simulink model "MMC_phase_hackathon_consensus_PWM_JABBAR_20260927"  (R2024b)
settings: Solver=FixedStepDiscrete  StartTime=t_init_sim  StopTime=sim_time  FixedStep=Ts  RelTol=1e-3
values from neighbouring files (symbols this model uses):
  a = 1    [script_MMC_phase_hackathon_consensus_PWM_JABBAR_20260927.m]
  C1low1_active = 1    [script_MMC_phase_hackathon_consensus_PWM_JABBAR_20260927.m]
  C2low1_active = 1    [script_MMC_phase_hackathon_consensus_PWM_JABBAR_20260927.m]
  C_bus = 4400e-6    (= 0.0044)    [script_MMC_phase_hackathon_consensus_PWM_JABBAR_20260927.m]
  C_M_extra = C_m-twist_high_side_C    [script_MMC_phase_hackathon_consensus_PWM_JABBAR_20260927.m]
  f0 = 50    [script_MMC_phase_hackathon_consensus_PWM_JABBAR_20260927.m]
  feeder_current_lower_rate_limit = -10    [script_MMC_phase_hackathon_consensus_PWM_JABBAR_20260927.m]    (also in twist_parameters.m = -500)
  feeder_current_tab = [0.328 0.217 0.162 0.132 0.109 0.094 0.083 0.075 0.068 0.062 0.058 0.054 ... (42 elements, 14x3)]    [feeder_current.mat]
  feeder_current_upper_rate_limit = 0.386/(20e-3)    (= 19.3)    [twist_parameters.m]
  is6VExternallySupplied = true    [script_MMC_phase_hackathon_consensus_PWM_JABBAR_20260927.m]
  isFeederJumperOpen = true    [script_MMC_phase_hackathon_consensus_PWM_JABBAR_20260927.m]
  L_arm = 100e-3    (= 0.1)    [script_MMC_phase_hackathon_consensus_PWM_JABBAR_20260927.m]
  m = 1    [script_MMC_phase_hackathon_consensus_PWM_JABBAR_20260927.m]
  power_losses = false    [script_MMC_phase_hackathon_consensus_PWM_JABBAR_20260927.m]
  R = 30    [script_MMC_phase_hackathon_consensus_PWM_JABBAR_20260927.m]
  R_arm = 0.2    [script_MMC_phase_hackathon_consensus_PWM_JABBAR_20260927.m]
  source_V = 0    [script_MMC_phase_hackathon_consensus_PWM_JABBAR_20260927.m]
  time_charge = 0.1    [script_MMC_phase_hackathon_consensus_PWM_JABBAR_20260927.m]
  time_decharge = 1.5    [script_MMC_phase_hackathon_consensus_PWM_JABBAR_20260927.m]
  Ts = 5e-7    (= 5e-07)    [script_MMC_phase_hackathon_consensus_PWM_JABBAR_20260927.m]
  twist_data_acquisition_delay = 50e-9    (= 5e-08)    [script_MMC_phase_hackathon_consensus_PWM_JABBAR_20260927.m]    (also in twist_parameters.m)
  twist_data_sampling_period = 1/twist_freq_data_sampling    (= 5e-05)    [script_MMC_phase_hackathon_consensus_PWM_JABBAR_20260927.m]    (also in twist_parameters.m)
  twist_dead_time = 200e-9    (= 2e-07)    [twist_parameters.m]
  twist_freq_switching = 200e3    (= 200000)    [twist_parameters.m]
  twist_high_side_adc_R = 1/(1/2e6 + 1/2e6 + 1/(330e3+5.6e3))    (= 251272.836178)    [twist_parameters.m]
  twist_high_side_C = 33e-6*4 + 4.7e-6*12    (= 0.0001884)    [twist_parameters.m]
  twist_high_side_feeder_R = 47e3+4.7e3    (= 51700)    [twist_parameters.m]
  twist_high_side_rC = 0.1    [twist_parameters.m]
  twist_low_side_adc_R = 150e3+470    (= 150470)    [twist_parameters.m]
  twist_low_side_C_ceramic = 3*4.7e-6    (= 1.41e-05)    [twist_parameters.m]
  twist_low_side_C_electrolytic = 47e-6    (= 4.7e-05)    [twist_parameters.m]
  twist_low_side_L = 33e-6    (= 3.3e-05)    [twist_parameters.m]
  twist_low_side_rC = 700e-3    (= 0.7)    [twist_parameters.m]
  twist_low_side_rL = 20e-3    (= 0.02)    [twist_parameters.m]
  twist_R_VCC = (tau_VCC/twist_high_side_C  - twist_high_side_rC)/(1-(tau_VCC/twist_high_side_C - twist_high_side_rC)/R_parallel)    (= 1110.74997822)    [twist_parameters.m]
  VDC = 48    [script_MMC_phase_hackathon_consensus_PWM_JABBAR_20260927.m]
undefined symbols (not defined in the file or in its folder): C_SM, feeder_current, gcbh, sps_rtmsupport, twist_low_side_lC
libraries: spsSeriesRLCBranchLib x135, spsTriangleGeneratorLib x60, spsMosfetLib x60, spsCurrentMeasurementLib x43, spsVoltageMeasurementLib x35, spsControlledCurrentSourceLib x30, spsDiodeLib x22, spsIdealSwitchLib x20, spsControlledVoltageSourceLib x1, spsGroundLib x1, spspowerguiLib x1
(part 17 of 19)

== system MMC_phase_hackathon_consensus_PWM_JABBAR_20260927/ /Subsystem/Subsystem1/Hardware M5/HRTimA_1/PWM Generator (2-Level)/Sampling/Sync Asymmetrical/Sample & Hold ==
  In : Inport
  Enable : EnablePort
  Out : Outport  VectorParamsAs1DForOutWhenUnconnected=off
  wires:
  In/1 -> Out/1

== system MMC_phase_hackathon_consensus_PWM_JABBAR_20260927/ /Subsystem/Subsystem1/Hardware M5/HRTimA_1/PWM Generator (2-Level)/Sampling/Sync Natural/Sync_NaturalSampling ==
  Uref : Inport  Interpolate=off
  wt : Inport  Port=2  Interpolate=off
  Gain1 : Gain  Gain=2/pi  SaturateOnIntegerOverflow=on  OutDataTypeStr=Inherit: Same as input  ParamDataTypeStr=Inherit: Same as input
  Gain4 : Gain  Gain=nF  SaturateOnIntegerOverflow=on  OutDataTypeStr=Inherit: Same as input  ParamDataTypeStr=Inherit: Same as input
  Trigonometric Function : Trigonometry  Operator=asin
  Trigonometric Function3 : Trigonometry
  Uref* : Outport  VectorParamsAs1DForOutWhenUnconnected=off
  Cr : Outport  Port=2  VectorParamsAs1DForOutWhenUnconnected=off
  wires:
  wt/1 -> Gain4/1
  Gain1/1 -> Cr/1
  Trigonometric Function/1 -> Gain1/1
  Trigonometric Function3/1 -> Trigonometric Function/1
  Gain4/1 -> Trigonometric Function3/1
  Uref/1 -> Uref*/1

== system MMC_phase_hackathon_consensus_PWM_JABBAR_20260927/ /Subsystem/Subsystem1/Hardware M5/HRTimA_1/PWM Generator (2-Level)/Sampling/Sync Symmetrical/Sync_SymmetricalSampling ==
  Uref : Inport  Interpolate=off
  wt : Inport  Port=2  Interpolate=off
  Add : Sum
  Constant3 : Constant
  Gain1 : Gain  Gain=2/pi  SaturateOnIntegerOverflow=on  OutDataTypeStr=Inherit: Same as input  ParamDataTypeStr=Inherit: Same as input
  Gain4 : Gain  Gain=nF  SaturateOnIntegerOverflow=on  OutDataTypeStr=Inherit: Same as input  ParamDataTypeStr=Inherit: Same as input
  Hit Crossing : HitCross  HitCrossingOffset=1e-9  HitCrossingDirection=falling
  Sample & Hold : Subsystem
  Trigonometric Function : Trigonometry  Operator=asin
  Trigonometric Function3 : Trigonometry
  Uref* : Outport  VectorParamsAs1DForOutWhenUnconnected=off
  Cr : Outport  Port=2  VectorParamsAs1DForOutWhenUnconnected=off
  wires:
  wt/1 -> Gain4/1
  Gain1/1 -> Cr/1, Add/1
  Trigonometric Function/1 -> Gain1/1
  Trigonometric Function3/1 -> Trigonometric Function/1
  Gain4/1 -> Trigonometric Function3/1
  Add/1 -> Hit Crossing/1
  Constant3/1 -> Add/2
  Hit Crossing/1 -> Sample & Hold/Enable
  Uref/1 -> Sample & Hold/1(In)
  Sample & Hold/1(Out) -> Uref*/1

== system MMC_phase_hackathon_consensus_PWM_JABBAR_20260927/ /Subsystem/Subsystem1/Hardware M5/HRTimA_1/PWM Generator (2-Level)/Sampling/Unsync Asymmetrical/Unsync_AsymmetricalSampling ==
  Uref : Inport  Interpolate=off
  Triangle Generator : spsTriangleGeneratorLib/Triangle Generator  Freq=sps.Fc  Phase=sps.Pc  Ts=Ts
  Zero-Order Hold : ZeroOrderHold  SampleTime=sps.SampleTimeZOH_AsymSampling
  Uref* : Outport  VectorParamsAs1DForOutWhenUnconnected=off
  Cr : Outport  Port=2  VectorParamsAs1DForOutWhenUnconnected=off
  wires:
  Triangle Generator/1 -> Cr/1
  Uref/1 -> Zero-Order Hold/1
  Zero-Order Hold/1 -> Uref*/1

== system MMC_phase_hackathon_consensus_PWM_JABBAR_20260927/ /Subsystem/Subsystem1/Hardware M5/HRTimA_1/PWM Generator (2-Level)/Sampling/Unsync Natural/Unsync_NaturalSampling ==
  Uref : Inport  Interpolate=off
  Triangle Generator : spsTriangleGeneratorLib/Triangle Generator  Freq=sps.Fc  Phase=sps.Pc  Ts=Ts
  Uref* : Outport  VectorParamsAs1DForOutWhenUnconnected=off
  Cr : Outport  Port=2  VectorParamsAs1DForOutWhenUnconnected=off
  wires:
  Triangle Generator/1 -> Cr/1
  Uref/1 -> Uref*/1

== system MMC_phase_hackathon_consensus_PWM_JABBAR_20260927/ /Subsystem/Subsystem1/Hardware M5/HRTimA_1/PWM Generator (2-Level)/Sampling/Unsync Symmetrical/Unsync_SymmetricalSampling ==
  Uref : Inport  Interpolate=off
  Triangle Generator : spsTriangleGeneratorLib/Triangle Generator  Freq=sps.Fc  Phase=sps.Pc  Ts=Ts
  Zero-Order Hold : ZeroOrderHold  SampleTime=sps.SampleTimeZOH_SymSampling
  Uref* : Outport  VectorParamsAs1DForOutWhenUnconnected=off
  Cr : Outport  Port=2  VectorParamsAs1DForOutWhenUnconnected=off
  wires:
  Triangle Generator/1 -> Cr/1
  Uref/1 -> Zero-Order Hold/1
  Zero-Order Hold/1 -> Uref*/1

== system MMC_phase_hackathon_consensus_PWM_JABBAR_20260927/ /Subsystem/Subsystem1/Hardware M5/HRTimA_2/PWM Generator (2-Level)/Sampling/Sync Asymmetrical/Sample & Hold ==
  In : Inport
  Enable : EnablePort
  Out : Outport  VectorParamsAs1DForOutWhenUnconnected=off
  wires:
  In/1 -> Out/1

== system MMC_phase_hackathon_consensus_PWM_JABBAR_20260927/ /Subsystem/Subsystem1/Hardware M5/HRTimA_2/PWM Generator (2-Level)/Sampling/Sync Natural/Sync_NaturalSampling ==
  Uref : Inport  Interpolate=off
  wt : Inport  Port=2  Interpolate=off
  Gain1 : Gain  Gain=2/pi  SaturateOnIntegerOverflow=on  OutDataTypeStr=Inherit: Same as input  ParamDataTypeStr=Inherit: Same as input
  Gain4 : Gain  Gain=nF  SaturateOnIntegerOverflow=on  OutDataTypeStr=Inherit: Same as input  ParamDataTypeStr=Inherit: Same as input
  Trigonometric Function : Trigonometry  Operator=asin
  Trigonometric Function3 : Trigonometry
  Uref* : Outport  VectorParamsAs1DForOutWhenUnconnected=off
  Cr : Outport  Port=2  VectorParamsAs1DForOutWhenUnconnected=off
  wires:
  wt/1 -> Gain4/1
  Gain1/1 -> Cr/1
  Trigonometric Function/1 -> Gain1/1
  Trigonometric Function3/1 -> Trigonometric Function/1
  Gain4/1 -> Trigonometric Function3/1
  Uref/1 -> Uref*/1

== system MMC_phase_hackathon_consensus_PWM_JABBAR_20260927/ /Subsystem/Subsystem1/Hardware M5/HRTimA_2/PWM Generator (2-Level)/Sampling/Sync Symmetrical/Sync_SymmetricalSampling ==
  Uref : Inport  Interpolate=off
  wt : Inport  Port=2  Interpolate=off
  Add : Sum
  Constant3 : Constant
  Gain1 : Gain  Gain=2/pi  SaturateOnIntegerOverflow=on  OutDataTypeStr=Inherit: Same as input  ParamDataTypeStr=Inherit: Same as input
  Gain4 : Gain  Gain=nF  SaturateOnIntegerOverflow=on  OutDataTypeStr=Inherit: Same as input  ParamDataTypeStr=Inherit: Same as input
  Hit Crossing : HitCross  HitCrossingOffset=1e-9  HitCrossingDirection=falling
  Sample & Hold : Subsystem
  Trigonometric Function : Trigonometry  Operator=asin
  Trigonometric Function3 : Trigonometry
  Uref* : Outport  VectorParamsAs1DForOutWhenUnconnected=off
  Cr : Outport  Port=2  VectorParamsAs1DForOutWhenUnconnected=off
  wires:
  wt/1 -> Gain4/1
  Gain1/1 -> Cr/1, Add/1
  Trigonometric Function/1 -> Gain1/1
  Trigonometric Function3/1 -> Trigonometric Function/1
  Gain4/1 -> Trigonometric Function3/1
  Add/1 -> Hit Crossing/1
  Constant3/1 -> Add/2
  Hit Crossing/1 -> Sample & Hold/Enable
  Uref/1 -> Sample & Hold/1(In)
  Sample & Hold/1(Out) -> Uref*/1

== system MMC_phase_hackathon_consensus_PWM_JABBAR_20260927/ /Subsystem/Subsystem1/Hardware M5/HRTimA_2/PWM Generator (2-Level)/Sampling/Unsync Asymmetrical/Unsync_AsymmetricalSampling ==
  Uref : Inport  Interpolate=off
  Triangle Generator : spsTriangleGeneratorLib/Triangle Generator  Freq=sps.Fc  Phase=sps.Pc  Ts=Ts
  Zero-Order Hold : ZeroOrderHold  SampleTime=sps.SampleTimeZOH_AsymSampling
  Uref* : Outport  VectorParamsAs1DForOutWhenUnconnected=off
  Cr : Outport  Port=2  VectorParamsAs1DForOutWhenUnconnected=off
  wires:
  Triangle Generator/1 -> Cr/1
  Uref/1 -> Zero-Order Hold/1
  Zero-Order Hold/1 -> Uref*/1

== system MMC_phase_hackathon_consensus_PWM_JABBAR_20260927/ /Subsystem/Subsystem1/Hardware M5/HRTimA_2/PWM Generator (2-Level)/Sampling/Unsync Natural/Unsync_NaturalSampling ==
  Uref : Inport  Interpolate=off
  Triangle Generator : spsTriangleGeneratorLib/Triangle Generator  Freq=sps.Fc  Phase=sps.Pc  Ts=Ts
  Uref* : Outport  VectorParamsAs1DForOutWhenUnconnected=off
  Cr : Outport  Port=2  VectorParamsAs1DForOutWhenUnconnected=off
  wires:
  Triangle Generator/1 -> Cr/1
  Uref/1 -> Uref*/1

== system MMC_phase_hackathon_consensus_PWM_JABBAR_20260927/ /Subsystem/Subsystem1/Hardware M5/HRTimA_2/PWM Generator (2-Level)/Sampling/Unsync Symmetrical/Unsync_SymmetricalSampling ==
  Uref : Inport  Interpolate=off
  Triangle Generator : spsTriangleGeneratorLib/Triangle Generator  Freq=sps.Fc  Phase=sps.Pc  Ts=Ts
  Zero-Order Hold : ZeroOrderHold  SampleTime=sps.SampleTimeZOH_SymSampling
  Uref* : Outport  VectorParamsAs1DForOutWhenUnconnected=off
  Cr : Outport  Port=2  VectorParamsAs1DForOutWhenUnconnected=off
  wires:
  Triangle Generator/1 -> Cr/1
  Uref/1 -> Zero-Order Hold/1
  Zero-Order Hold/1 -> Uref*/1

== system MMC_phase_hackathon_consensus_PWM_JABBAR_20260927/ /Subsystem/Subsystem/Hardware M1/HRTimA_1/PWM Generator (2-Level)/Sampling/Sync Symmetrical/Sync_SymmetricalSampling/Sample & Hold ==
  In : Inport
  Enable : EnablePort
  Out : Outport  VectorParamsAs1DForOutWhenUnconnected=off
  wires:
  In/1 -> Out/1

== system MMC_phase_hackathon_consensus_PWM_JABBAR_20260927/ /Subsystem/Subsystem/Hardware M1/HRTimA_2/PWM Generator (2-Level)/Sampling/Sync Symmetrical/Sync_SymmetricalSampling/Sample & Hold ==
  In : Inport
  Enable : EnablePort
  Out : Outport  VectorParamsAs1DForOutWhenUnconnected=off
  wires:
  In/1 -> Out/1

== system MMC_phase_hackathon_consensus_PWM_JABBAR_20260927/ /Subsystem/Subsystem/Hardware M2/HRTimA_1/PWM Generator (2-Level)/Sampling/Sync Symmetrical/Sync_SymmetricalSampling/Sample & Hold ==
  In : Inport
  Enable : EnablePort
  Out : Outport  VectorParamsAs1DForOutWhenUnconnected=off
  wires:
  In/1 -> Out/1

== system MMC_phase_hackathon_consensus_PWM_JABBAR_20260927/ /Subsystem/Subsystem/Hardware M2/HRTimA_2/PWM Generator (2-Level)/Sampling/Sync Symmetrical/Sync_SymmetricalSampling/Sample & Hold ==
  In : Inport
  Enable : EnablePort
  Out : Outport  VectorParamsAs1DForOutWhenUnconnected=off
  wires:
  In/1 -> Out/1

== system MMC_phase_hackathon_consensus_PWM_JABBAR_20260927/ /Subsystem/Subsystem/Hardware M3/HRTimA_1/PWM Generator (2-Level)/Sampling/Sync Symmetrical/Sync_SymmetricalSampling/Sample & Hold ==
  In : Inport
  Enable : EnablePort
  Out : Outport  VectorParamsAs1DForOutWhenUnconnected=off
  wires:
  In/1 -> Out/1

== system MMC_phase_hackathon_consensus_PWM_JABBAR_20260927/ /Subsystem/Subsystem/Hardware M3/HRTimA_2/PWM Generator (2-Level)/Sampling/Sync Symmetrical/Sync_SymmetricalSampling/Sample & Hold ==
  In : Inport
  Enable : EnablePort
  Out : Outport  VectorParamsAs1DForOutWhenUnconnected=off
  wires:
  In/1 -> Out/1

== system MMC_phase_hackathon_consensus_PWM_JABBAR_20260927/ /Subsystem/Subsystem/Hardware M4/HRTimA_1/PWM Generator (2-Level)/Sampling/Sync Symmetrical/Sync_SymmetricalSampling/Sample & Hold ==
  In : Inport
  Enable : EnablePort
  Out : Outport  VectorParamsAs1DForOutWhenUnconnected=off
  wires:
  In/1 -> Out/1

== system MMC_phase_hackathon_consensus_PWM_JABBAR_20260927/ /Subsystem/Subsystem/Hardware M4/HRTimA_2/PWM Generator (2-Level)/Sampling/Sync Symmetrical/Sync_SymmetricalSampling/Sample & Hold ==
  In : Inport
  Enable : EnablePort
  Out : Outport  VectorParamsAs1DForOutWhenUnconnected=off
  wires:
  In/1 -> Out/1

== system MMC_phase_hackathon_consensus_PWM_JABBAR_20260927/ /Subsystem/Subsystem/Hardware M5/HRTimA_1/PWM Generator (2-Level)/Sampling/Sync Symmetrical/Sync_SymmetricalSampling/Sample & Hold ==
  In : Inport
  Enable : EnablePort
  Out : Outport  VectorParamsAs1DForOutWhenUnconnected=off
  wires:
  In/1 -> Out/1

== system MMC_phase_hackathon_consensus_PWM_JABBAR_20260927/ /Subsystem/Subsystem/Hardware M5/HRTimA_2/PWM Generator (2-Level)/Sampling/Sync Symmetrical/Sync_SymmetricalSampling/Sample & Hold ==
  In : Inport
  Enable : EnablePort
  Out : Outport  VectorParamsAs1DForOutWhenUnconnected=off
  wires:
  In/1 -> Out/1

== system MMC_phase_hackathon_consensus_PWM_JABBAR_20260927/ /Subsystem/Subsystem1/Hardware M1/HRTimA_1/PWM Generator (2-Level)/Sampling/Sync Symmetrical/Sync_SymmetricalSampling/Sample & Hold ==
  In : Inport
  Enable : EnablePort
  Out : Outport  VectorParamsAs1DForOutWhenUnconnected=off
  wires:
  In/1 -> Out/1

== system MMC_phase_hackathon_consensus_PWM_JABBAR_20260927/ /Subsystem/Subsystem1/Hardware M1/HRTimA_2/PWM Generator (2-Level)/Sampling/Sync Symmetrical/Sync_SymmetricalSampling/Sample & Hold ==
  In : Inport
  Enable : EnablePort
  Out : Outport  VectorParamsAs1DForOutWhenUnconnected=off
  wires:
  In/1 -> Out/1

== system MMC_phase_hackathon_consensus_PWM_JABBAR_20260927/ /Subsystem/Subsystem1/Hardware M2/HRTimA_1/PWM Generator (2-Level)/Sampling/Sync Symmetrical/Sync_SymmetricalSampling/Sample & Hold ==
  In : Inport
  Enable : EnablePort
  Out : Outport  VectorParamsAs1DForOutWhenUnconnected=off
  wires:
  In/1 -> Out/1

== system MMC_phase_hackathon_consensus_PWM_JABBAR_20260927/ /Subsystem/Subsystem1/Hardware M2/HRTimA_2/PWM Generator (2-Level)/Sampling/Sync Symmetrical/Sync_SymmetricalSampling/Sample & Hold ==
  In : Inport
  Enable : EnablePort
  Out : Outport  VectorParamsAs1DForOutWhenUnconnected=off
  wires:
  In/1 -> Out/1

== system MMC_phase_hackathon_consensus_PWM_JABBAR_20260927/ /Subsystem/Subsystem1/Hardware M3/HRTimA_1/PWM Generator (2-Level)/Sampling/Sync Symmetrical/Sync_SymmetricalSampling/Sample & Hold ==
  In : Inport
  Enable : EnablePort
  Out : Outport  VectorParamsAs1DForOutWhenUnconnected=off
  wires:
  In/1 -> Out/1

== system MMC_phase_hackathon_consensus_PWM_JABBAR_20260927/ /Subsystem/Subsystem1/Hardware M3/HRTimA_2/PWM Generator (2-Level)/Sampling/Sync Symmetrical/Sync_SymmetricalSampling/Sample & Hold ==
  In : Inport
  Enable : EnablePort
  Out : Outport  VectorParamsAs1DForOutWhenUnconnected=off
  wires:
  In/1 -> Out/1

== system MMC_phase_hackathon_consensus_PWM_JABBAR_20260927/ /Subsystem/Subsystem1/Hardware M4/HRTimA_1/PWM Generator (2-Level)/Sampling/Sync Symmetrical/Sync_SymmetricalSampling/Sample & Hold ==
  In : Inport
  Enable : EnablePort
  Out : Outport  VectorParamsAs1DForOutWhenUnconnected=off
  wires:
  In/1 -> Out/1

== system MMC_phase_hackathon_consensus_PWM_JABBAR_20260927/ /Subsystem/Subsystem1/Hardware M4/HRTimA_2/PWM Generator (2-Level)/Sampling/Sync Symmetrical/Sync_SymmetricalSampling/Sample & Hold ==
  In : Inport
  Enable : EnablePort
  Out : Outport  VectorParamsAs1DForOutWhenUnconnected=off
  wires:
  In/1 -> Out/1

== system MMC_phase_hackathon_consensus_PWM_JABBAR_20260927/ /Subsystem/Subsystem1/Hardware M5/HRTimA_1/PWM Generator (2-Level)/Sampling/Sync Symmetrical/Sync_SymmetricalSampling/Sample & Hold ==
  In : Inport
  Enable : EnablePort
  Out : Outport  VectorParamsAs1DForOutWhenUnconnected=off
  wires:
  In/1 -> Out/1

== system MMC_phase_hackathon_consensus_PWM_JABBAR_20260927/ /Subsystem/Subsystem1/Hardware M5/HRTimA_2/PWM Generator (2-Level)/Sampling/Sync Symmetrical/Sync_SymmetricalSampling/Sample & Hold ==
  In : Inport
  Enable : EnablePort
  Out : Outport  VectorParamsAs1DForOutWhenUnconnected=off
  wires:
  In/1 -> Out/1

== matlab function MMC_phase_hackathon_consensus_PWM_JABBAR_20260927/ /Subsystem/Subsystem/Hardware M3/Feeder block/MATLAB Function ==
  data: i_feeder input; vC input; isfeederdisabled input; active_1 input; y output; Q_VCC output
function [y,Q_VCC]  = feeder_characteristics(i_feeder,vC,isfeederdisabled,active_1)

if(isfeederdisabled == 1)
    if(vC>=9.7)
        y = 11.2e-3;
        Q_VCC = 0;
    elseif(vC>=8.9 && vC < 9.7)
        if(active_1 == true)
            y = 11.2e-3;
            Q_VCC = 0;
        else
            y = 0;
            Q_VCC = 1;
        end
    else
        y = 0;
        Q_VCC = 1;
    end
else
    if(vC>=9.7)
        y = i_feeder;
        Q_VCC = 0;
    elseif(vC>=8.9 && vC < 9.7)
        if(active_1 == true)
            y = i_feeder;
            Q_VCC = 0;
        else
            y = 0;
            Q_VCC = 1;
        end
    else
        y = 0;
        Q_VCC = 1;
    end
end

== matlab function MMC_phase_hackathon_consensus_PWM_JABBAR_20260927/ /Subsystem/Subsystem/Hardware M3/Power losses branch 1/Branch DT loss ==
  data: twist_FET_Pdt output; ILow input
function twist_FET_Pdt = powerLossesDeadTime(ILow)
    %Twist gate power losses
    twist_freq_switching = 200e3;
    twist_FET_Vf = 1.2;
    twist_FET_tDr = 10e-9;
    twist_FET_tDf = 0;

    twist_FET_Pdt = twist_FET_Vf*ILow*(twist_FET_tDr+twist_FET_tDf)*twist_freq_switching;
end

== matlab function MMC_phase_hackathon_consensus_PWM_JABBAR_20260927/ /Sinus Modulation + Sorting Algorithm/Subsystem1/Subsystem/MATLAB Function3 ==
  data: sm_id input; m_arm input; gate_signal output; i_arm input; Vc_arm input; Vc_prev input; Vc_next input; N input
function gate_signal = hb_sm_local_ctrl_neighbor(sm_id, m_arm, i_arm, Vc_arm, Vc_prev, Vc_next, N)
%#codegen
% =========================================================
% LOCAL CONSENSUS BALANCING (v9) - matched to existing PSC-PWM hardware
%
% Implements the user's hb_sm_local_ctrl_consensus algorithm:
%   - Consensus balancing with neighbour-only Vref (distributed)
%   - Voltage deadband suppresses correction near steady state
%   - tanh(i_arm/Iscale) smooth sign avoids zero-current discontinuity
%
% Output is m_i as a continuous duty in [0, 1]. The downstream PWM
% Generator block carries the phase-shifted carrier (Phase = sps.Pc,
% configured per-SM in the parameter file) and produces the actual
% gate signal -- so we get phase-shifted PWM switching at the arm
% level without needing to generate a carrier in software.
%
% Inputs N and Vc_arm beyond v_current are unused but kept in the
% signature so the parent subsystem wiring is unchanged.
% =========================================================

% --- 1. PARAMETERS (verbatim from user spec) ---
k_v      = double(0.2);    % Balancing gain (1/V)
deadband = double(0.1);    % Voltage-error deadband (V)
Iscale   = double(1.0);    % Current scaling for tanh smoothing (A)

% --- 2. CONSENSUS BALANCING WITH LOCAL NEIGHBOUR REFERENCE ---
Vc_i = double(Vc_arm(sm_id));

% err: deviation of this SM from its immediate neighbours.
%   err > 0  -> this SM is BELOW neighbour average -> needs more charge
%   err < 0  -> this SM is ABOVE neighbour average -> needs less charge
err = double(0.5 * (Vc_prev + Vc_next)) - Vc_i;

% Deadband: ignore micro-imbalance near steady state.
if abs(err) < deadband
    err = 0.0;
end

% dir: smooth current-direction signal via tanh.
% Avoids the discontinuity of sign() near zero current crossings.
dir = tanh(double(i_arm) / Iscale);

% dm: balancing correction on the modulation index
dm = k_v * err * dir;

% m_i: per-SM corrected modulation index, clamped to [0, 1]
m_i = min(max(double(m_arm) + dm, 0.0), 1.0);

% --- 3. OUTPUT: duty cycle for the downstream phase-shifted PWM block ---
gate_signal = double(m_i);

end

== matlab function MMC_phase_hackathon_consensus_PWM_JABBAR_20260927/ /Subsystem/Subsystem/Hardware M1/Feeder block/MATLAB Function ==
  data: i_feeder input; vC input; isfeederdisabled input; active_1 input; y output; Q_VCC output
function [y,Q_VCC]  = feeder_characteristics(i_feeder,vC,isfeederdisabled,active_1)

if(isfeederdisabled == 1)
    if(vC>=9.7)
        y = 11.2e-3;
        Q_VCC = 0;
    elseif(vC>=8.9 && vC < 9.7)
        if(active_1 == true)
            y = 11.2e-3;
            Q_VCC = 0;
        else
            y = 0;
            Q_VCC = 1;
        end
    else
        y = 0;
        Q_VCC = 1;
    end
else
    if(vC>=9.7)
        y = i_feeder;
        Q_VCC = 0;
    elseif(vC>=8.9 && vC < 9.7)
        if(active_1 == true)
            y = i_feeder;
            Q_VCC = 0;
        else
            y = 0;
            Q_VCC = 1;
        end
    else
        y = 0;
        Q_VCC = 1;
    end
end

== matlab function MMC_phase_hackathon_consensus_PWM_JABBAR_20260927/ /Sinus Modulation + Sorting Algorithm/Subsystem1/Subsystem/MATLAB Function1 ==
  data: Vc_arm input; i input; Vc_prev output; Vc_next output
function [Vc_prev, Vc_next] = get_neighbors(Vc_arm, i)
%#codegen
% Returns the capacitor voltages of the previous and next (circular) neighbors.
% Hardcoded strictly for N = 5 sub-modules per arm.

N = 5; 

% MATHEMATICAL CIRCULAR INDEXING FOR N = 5:
% If i=1 -> idx_prev = 5, idx_next = 2
% If i=5 -> idx_prev = 4, idx_next = 1

idx_prev = mod(i - 2, N) + 1;
idx_next = mod(i, N) + 1;

Vc_prev = Vc_arm(idx_prev);
Vc_next = Vc_arm(idx_next);

end

== matlab function MMC_phase_hackathon_consensus_PWM_JABBAR_20260927/ /Subsystem/Subsystem/Hardware M1/Power losses branch 1/Branch DT loss ==
  data: twist_FET_Pdt output; ILow input
function twist_FET_Pdt = powerLossesDeadTime(ILow)
    %Twist gate power losses
    twist_freq_switching = 200e3;
    twist_FET_Vf = 1.2;
    twist_FET_tDr = 10e-9;
    twist_FET_tDf = 0;

    twist_FET_Pdt = twist_FET_Vf*ILow*(twist_FET_tDr+twist_FET_tDf)*twist_freq_switching;
end

== matlab function MMC_phase_hackathon_consensus_PWM_JABBAR_20260927/ /Subsystem/Subsystem/Hardware M1/Power losses branch 1/Branch cond loss ==
  data: twist_FET_Pcond output; VHigh input; VLow input; ILow input
function twist_FET_Pcond = powerLossesCond(VHigh, VLow, ILow)
    %Twist conduction power losses
    twist_FET_Ron = 0.025;

    twist_FET_PcondH = pow2(ILow)*twist_FET_Ron*(VLow/VHigh);
    twist_FET_PcondL = pow2(ILow)*twist_FET_Ron*(1 - VLow/VHigh);

    twist_FET_Pcond = twist_FET_PcondH + twist_FET_PcondL;
end

== matlab function MMC_phase_hackathon_consensus_PWM_JABBAR_20260927/ /Subsystem/Subsystem/Hardware M1/Power losses branch 1/Branch gate loss ==
  data: twist_FET_Pg output
function twist_FET_Pg = powerLossesGate()
    %Twist gate power losses
    twist_freq_switching = 200e3;
    twist_FET_QgH = 31e-9;
    twist_FET_QgL = 31e-9;
    twist_FET_Vgs = 11;

    twist_FET_Pg = (twist_FET_QgH + twist_FET_QgL)*twist_FET_Vgs*twist_freq_switching;
end

== matlab function MMC_phase_hackathon_consensus_PWM_JABBAR_20260927/ /Subsystem/Subsystem/Hardware M1/Power losses branch 1/Branch switching loss ==
  data: VHigh input; twist_FET_Psw output; ILow input
function twist_FET_Psw = powerLossesSwitch(VHigh, ILow)
    %Twist switch power losses
    twist_freq_switching = 200e3;
    twist_FET_trise = 17e-9;
    twist_FET_tfall = 9e-9;

    twist_FET_Psw = 1/2*VHigh*ILow*twist_freq_switching*(twist_FET_trise + twist_FET_tfall);
end

== matlab function MMC_phase_hackathon_consensus_PWM_JABBAR_20260927/ /Subsystem/Subsystem/Hardware M1/Power losses branch 2/Branch DT loss ==
  data: twist_FET_Pdt output; ILow input
function twist_FET_Pdt = powerLossesDeadTime(ILow)
    %Twist gate power losses
    twist_freq_switching = 200e3;
    twist_FET_Vf = 1.2;
    twist_FET_tDr = 10e-9;
    twist_FET_tDf = 0;

    twist_FET_Pdt = twist_FET_Vf*ILow*(twist_FET_tDr+twist_FET_tDf)*twist_freq_switching;
end

== matlab function MMC_phase_hackathon_consensus_PWM_JABBAR_20260927/ /Subsystem/Subsystem/Hardware M1/Power losses branch 2/Branch cond loss ==
  data: twist_FET_Pcond output; VHigh input; VLow input; ILow input
function twist_FET_Pcond = powerLossesCond(VHigh, VLow, ILow)
    %Twist conduction power losses
    twist_FET_Ron = 0.025;

    twist_FET_PcondH = pow2(ILow)*twist_FET_Ron*(VLow/VHigh);
    twist_FET_PcondL = pow2(ILow)*twist_FET_Ron*(1 - VLow/VHigh);

    twist_FET_Pcond = twist_FET_PcondH + twist_FET_PcondL;
end

== matlab function MMC_phase_hackathon_consensus_PWM_JABBAR_20260927/ /Subsystem/Subsystem/Hardware M1/Power losses branch 2/Branch gate loss ==
  data: twist_FET_Pg output
function twist_FET_Pg = powerLossesGate()
    %Twist gate power losses
    twist_freq_switching = 200e3;
    twist_FET_QgH = 31e-9;
    twist_FET_QgL = 31e-9;
    twist_FET_Vgs = 11;

    twist_FET_Pg = (twist_FET_QgH + twist_FET_QgL)*twist_FET_Vgs*twist_freq_switching;
end

== matlab function MMC_phase_hackathon_consensus_PWM_JABBAR_20260927/ /Subsystem/Subsystem/Hardware M1/Power losses branch 2/Branch switching loss ==
  data: VHigh input; twist_FET_Psw output; ILow input
function twist_FET_Psw = powerLossesSwitch(VHigh, ILow)
    %Twist switch power losses
    twist_freq_switching = 200e3;
    twist_FET_trise = 17e-9;
    twist_FET_tfall = 9e-9;

    twist_FET_Psw = 1/2*VHigh*ILow*twist_freq_switching*(twist_FET_trise + twist_FET_tfall);
end

== matlab function MMC_phase_hackathon_consensus_PWM_JABBAR_20260927/ /Subsystem/Subsystem/Hardware M3/Power losses branch 1/Branch cond loss ==
  data: twist_FET_Pcond output; VHigh input; VLow input; ILow input
function twist_FET_Pcond = powerLossesCond(VHigh, VLow, ILow)
    %Twist conduction power losses
    twist_FET_Ron = 0.025;

    twist_FET_PcondH = pow2(ILow)*twist_FET_Ron*(VLow/VHigh);
    twist_FET_PcondL = pow2(ILow)*twist_FET_Ron*(1 - VLow/VHigh);

    twist_FET_Pcond = twist_FET_PcondH + twist_FET_PcondL;
end

== matlab function MMC_phase_hackathon_consensus_PWM_JABBAR_20260927/ /Subsystem/Subsystem/Hardware M3/Power losses branch 1/Branch gate loss ==
  data: twist_FET_Pg output
function twist_FET_Pg = powerLossesGate()
    %Twist gate power losses
    twist_freq_switching = 200e3;
    twist_FET_QgH = 31e-9;
    twist_FET_QgL = 31e-9;
    twist_FET_Vgs = 11;

    twist_FET_Pg = (twist_FET_QgH + twist_FET_QgL)*twist_FET_Vgs*twist_freq_switching;
end

== matlab function MMC_phase_hackathon_consensus_PWM_JABBAR_20260927/ /Subsystem/Subsystem/Hardware M3/Power losses branch 1/Branch switching loss ==
  data: VHigh input; twist_FET_Psw output; ILow input
function twist_FET_Psw = powerLossesSwitch(VHigh, ILow)
    %Twist switch power losses
    twist_freq_switching = 200e3;
    twist_FET_trise = 17e-9;
    twist_FET_tfall = 9e-9;

    twist_FET_Psw = 1/2*VHigh*ILow*twist_freq_switching*(twist_FET_trise + twist_FET_tfall);
end

== matlab function MMC_phase_hackathon_consensus_PWM_JABBAR_20260927/ /Subsystem/Subsystem/Hardware M3/Power losses branch 2/Branch DT loss ==
  data: twist_FET_Pdt output; ILow input
function twist_FET_Pdt = powerLossesDeadTime(ILow)
    %Twist gate power losses
    twist_freq_switching = 200e3;
    twist_FET_Vf = 1.2;
    twist_FET_tDr = 10e-9;
    twist_FET_tDf = 0;

    twist_FET_Pdt = twist_FET_Vf*ILow*(twist_FET_tDr+twist_FET_tDf)*twist_freq_switching;
end

== matlab function MMC_phase_hackathon_consensus_PWM_JABBAR_20260927/ /Subsystem/Subsystem/Hardware M3/Power losses branch 2/Branch cond loss ==
  data: twist_FET_Pcond output; VHigh input; VLow input; ILow input
function twist_FET_Pcond = powerLossesCond(VHigh, VLow, ILow)
    %Twist conduction power losses
    twist_FET_Ron = 0.025;

    twist_FET_PcondH = pow2(ILow)*twist_FET_Ron*(VLow/VHigh);
    twist_FET_PcondL = pow2(ILow)*twist_FET_Ron*(1 - VLow/VHigh);

    twist_FET_Pcond = twist_FET_PcondH + twist_FET_PcondL;
end

== matlab function MMC_phase_hackathon_consensus_PWM_JABBAR_20260927/ /Subsystem/Subsystem/Hardware M3/Power losses branch 2/Branch gate loss ==
  data: twist_FET_Pg output
function twist_FET_Pg = powerLossesGate()
    %Twist gate power losses
    twist_freq_switching = 200e3;
    twist_FET_QgH = 31e-9;
    twist_FET_QgL = 31e-9;
    twist_FET_Vgs = 11;

    twist_FET_Pg = (twist_FET_QgH + twist_FET_QgL)*twist_FET_Vgs*twist_freq_switching;
end

== matlab function MMC_phase_hackathon_consensus_PWM_JABBAR_20260927/ /Subsystem/Subsystem/Hardware M3/Power losses branch 2/Branch switching loss ==
  data: VHigh input; twist_FET_Psw output; ILow input
function twist_FET_Psw = powerLossesSwitch(VHigh, ILow)
    %Twist switch power losses
    twist_freq_switching = 200e3;
    twist_FET_trise = 17e-9;
    twist_FET_tfall = 9e-9;

    twist_FET_Psw = 1/2*VHigh*ILow*twist_freq_switching*(twist_FET_trise + twist_FET_tfall);
end

== matlab function MMC_phase_hackathon_consensus_PWM_JABBAR_20260927/ /Subsystem/Subsystem/Hardware M4/Feeder block/MATLAB Function ==
  data: i_feeder input; vC input; isfeederdisabled input; active_1 input; y output; Q_VCC output
function [y,Q_VCC]  = feeder_characteristics(i_feeder,vC,isfeederdisabled,active_1)

if(isfeederdisabled == 1)
    if(vC>=9.7)
        y = 11.2e-3;
        Q_VCC = 0;
    elseif(vC>=8.9 && vC < 9.7)
        if(active_1 == true)
            y = 11.2e-3;
            Q_VCC = 0;
        else
            y = 0;
            Q_VCC = 1;
        end
    else
        y = 0;
        Q_VCC = 1;
    end
else
    if(vC>=9.7)
        y = i_feeder;
        Q_VCC = 0;
    elseif(vC>=8.9 && vC < 9.7)
        if(active_1 == true)
            y = i_feeder;
            Q_VCC = 0;
        else
            y = 0;
            Q_VCC = 1;
        end
    else
        y = 0;
        Q_VCC = 1;
    end
end

== matlab function MMC_phase_hackathon_consensus_PWM_JABBAR_20260927/ /Subsystem/Subsystem/Hardware M4/Power losses branch 1/Branch DT loss ==
  data: twist_FET_Pdt output; ILow input
function twist_FET_Pdt = powerLossesDeadTime(ILow)
    %Twist gate power losses
    twist_freq_switching = 200e3;
    twist_FET_Vf = 1.2;
    twist_FET_tDr = 10e-9;
    twist_FET_tDf = 0;

    twist_FET_Pdt = twist_FET_Vf*ILow*(twist_FET_tDr+twist_FET_tDf)*twist_freq_switching;
end

== matlab function MMC_phase_hackathon_consensus_PWM_JABBAR_20260927/ /Subsystem/Subsystem/Hardware M4/Power losses branch 1/Branch cond loss ==
  data: twist_FET_Pcond output; VHigh input; VLow input; ILow input
function twist_FET_Pcond = powerLossesCond(VHigh, VLow, ILow)
    %Twist conduction power losses
    twist_FET_Ron = 0.025;

    twist_FET_PcondH = pow2(ILow)*twist_FET_Ron*(VLow/VHigh);
    twist_FET_PcondL = pow2(ILow)*twist_FET_Ron*(1 - VLow/VHigh);

    twist_FET_Pcond = twist_FET_PcondH + twist_FET_PcondL;
end

== matlab function MMC_phase_hackathon_consensus_PWM_JABBAR_20260927/ /Subsystem/Subsystem/Hardware M4/Power losses branch 1/Branch gate loss ==
  data: twist_FET_Pg output
function twist_FET_Pg = powerLossesGate()
    %Twist gate power losses
    twist_freq_switching = 200e3;
    twist_FET_QgH = 31e-9;
    twist_FET_QgL = 31e-9;
    twist_FET_Vgs = 11;

    twist_FET_Pg = (twist_FET_QgH + twist_FET_QgL)*twist_FET_Vgs*twist_freq_switching;
end

== matlab function MMC_phase_hackathon_consensus_PWM_JABBAR_20260927/ /Subsystem/Subsystem/Hardware M4/Power losses branch 1/Branch switching loss ==
  data: VHigh input; twist_FET_Psw output; ILow input
function twist_FET_Psw = powerLossesSwitch(VHigh, ILow)
    %Twist switch power losses
    twist_freq_switching = 200e3;
    twist_FET_trise = 17e-9;
    twist_FET_tfall = 9e-9;

    twist_FET_Psw = 1/2*VHigh*ILow*twist_freq_switching*(twist_FET_trise + twist_FET_tfall);
end

== matlab function MMC_phase_hackathon_consensus_PWM_JABBAR_20260927/ /Subsystem/Subsystem/Hardware M4/Power losses branch 2/Branch DT loss ==
  data: twist_FET_Pdt output; ILow input
function twist_FET_Pdt = powerLossesDeadTime(ILow)
    %Twist gate power losses
    twist_freq_switching = 200e3;
    twist_FET_Vf = 1.2;
    twist_FET_tDr = 10e-9;
    twist_FET_tDf = 0;

    twist_FET_Pdt = twist_FET_Vf*ILow*(twist_FET_tDr+twist_FET_tDf)*twist_freq_switching;
end

== matlab function MMC_phase_hackathon_consensus_PWM_JABBAR_20260927/ /Subsystem/Subsystem/Hardware M4/Power losses branch 2/Branch cond loss ==
  data: twist_FET_Pcond output; VHigh input; VLow input; ILow input
function twist_FET_Pcond = powerLossesCond(VHigh, VLow, ILow)
    %Twist conduction power losses
    twist_FET_Ron = 0.025;

    twist_FET_PcondH = pow2(ILow)*twist_FET_Ron*(VLow/VHigh);
    twist_FET_PcondL = pow2(ILow)*twist_FET_Ron*(1 - VLow/VHigh);

    twist_FET_Pcond = twist_FET_PcondH + twist_FET_PcondL;
end

== matlab function MMC_phase_hackathon_consensus_PWM_JABBAR_20260927/ /Subsystem/Subsystem/Hardware M4/Power losses branch 2/Branch gate loss ==
  data: twist_FET_Pg output
function twist_FET_Pg = powerLossesGate()
    %Twist gate power losses
    twist_freq_switching = 200e3;
    twist_FET_QgH = 31e-9;
    twist_FET_QgL = 31e-9;
    twist_FET_Vgs = 11;

    twist_FET_Pg = (twist_FET_QgH + twist_FET_QgL)*twist_FET_Vgs*twist_freq_switching;
end

== matlab function MMC_phase_hackathon_consensus_PWM_JABBAR_20260927/ /Subsystem/Subsystem/Hardware M4/Power losses branch 2/Branch switching loss ==
  data: VHigh input; twist_FET_Psw output; ILow input
function twist_FET_Psw = powerLossesSwitch(VHigh, ILow)
    %Twist switch power losses
    twist_freq_switching = 200e3;
    twist_FET_trise = 17e-9;
    twist_FET_tfall = 9e-9;

    twist_FET_Psw = 1/2*VHigh*ILow*twist_freq_switching*(twist_FET_trise + twist_FET_tfall);
end

== matlab function MMC_phase_hackathon_consensus_PWM_JABBAR_20260927/ /Subsystem/Subsystem/Hardware M5/Feeder block/MATLAB Function ==
  data: i_feeder input; vC input; isfeederdisabled input; active_1 input; y output; Q_VCC output
function [y,Q_VCC]  = feeder_characteristics(i_feeder,vC,isfeederdisabled,active_1)

if(isfeederdisabled == 1)
    if(vC>=9.7)
        y = 11.2e-3;
        Q_VCC = 0;
    elseif(vC>=8.9 && vC < 9.7)
        if(active_1 == true)
            y = 11.2e-3;
            Q_VCC = 0;
        else
            y = 0;
            Q_VCC = 1;
        end
    else
        y = 0;
        Q_VCC = 1;
    end
else
    if(vC>=9.7)
        y = i_feeder;
        Q_VCC = 0;
    elseif(vC>=8.9 && vC < 9.7)
        if(active_1 == true)
            y = i_feeder;
            Q_VCC = 0;
        else
            y = 0;
            Q_VCC = 1;
        end
    else
        y = 0;
        Q_VCC = 1;
    end
end

== matlab function MMC_phase_hackathon_consensus_PWM_JABBAR_20260927/ /Subsystem/Subsystem/Hardware M5/Power losses branch 1/Branch DT loss ==
  data: twist_FET_Pdt output; ILow input
function twist_FET_Pdt = powerLossesDeadTime(ILow)
    %Twist gate power losses
    twist_freq_switching = 200e3;
    twist_FET_Vf = 1.2;
    twist_FET_tDr = 10e-9;
    twist_FET_tDf = 0;

    twist_FET_Pdt = twist_FET_Vf*ILow*(twist_FET_tDr+twist_FET_tDf)*twist_freq_switching;
end

== matlab function MMC_phase_hackathon_consensus_PWM_JABBAR_20260927/ /Subsystem/Subsystem/Hardware M2/Feeder block/MATLAB Function ==
  data: i_feeder input; vC input; isfeederdisabled input; active_1 input; y output; Q_VCC output
function [y,Q_VCC]  = feeder_characteristics(i_feeder,vC,isfeederdisabled,active_1)

if(isfeederdisabled == 1)
    if(vC>=9.7)
        y = 11.2e-3;
        Q_VCC = 0;
    elseif(vC>=8.9 && vC < 9.7)
        if(active_1 == true)
            y = 11.2e-3;
            Q_VCC = 0;
        else
            y = 0;
            Q_VCC = 1;
        end
    else
        y = 0;
        Q_VCC = 1;
    end
else
    if(vC>=9.7)
        y = i_feeder;
        Q_VCC = 0;
    elseif(vC>=8.9 && vC < 9.7)
        if(active_1 == true)
            y = i_feeder;
            Q_VCC = 0;
        else
            y = 0;
            Q_VCC = 1;
        end
    else
        y = 0;
        Q_VCC = 1;
    end
end

== matlab function MMC_phase_hackathon_consensus_PWM_JABBAR_20260927/ /Subsystem/Subsystem/Hardware M5/Power losses branch 1/Branch cond loss ==
  data: twist_FET_Pcond output; VHigh input; VLow input; ILow input
function twist_FET_Pcond = powerLossesCond(VHigh, VLow, ILow)
    %Twist conduction power losses
    twist_FET_Ron = 0.025;

    twist_FET_PcondH = pow2(ILow)*twist_FET_Ron*(VLow/VHigh);
    twist_FET_PcondL = pow2(ILow)*twist_FET_Ron*(1 - VLow/VHigh);

    twist_FET_Pcond = twist_FET_PcondH + twist_FET_PcondL;
end

== matlab function MMC_phase_hackathon_consensus_PWM_JABBAR_20260927/ /Subsystem/Subsystem/Hardware M5/Power losses branch 1/Branch gate loss ==
  data: twist_FET_Pg output
function twist_FET_Pg = powerLossesGate()
    %Twist gate power losses
    twist_freq_switching = 200e3;
    twist_FET_QgH = 31e-9;
    twist_FET_QgL = 31e-9;
    twist_FET_Vgs = 11;

    twist_FET_Pg = (twist_FET_QgH + twist_FET_QgL)*twist_FET_Vgs*twist_freq_switching;
end

== matlab function MMC_phase_hackathon_consensus_PWM_JABBAR_20260927/ /Subsystem/Subsystem/Hardware M5/Power losses branch 1/Branch switching loss ==
  data: VHigh input; twist_FET_Psw output; ILow input
function twist_FET_Psw = powerLossesSwitch(VHigh, ILow)
    %Twist switch power losses
    twist_freq_switching = 200e3;
    twist_FET_trise = 17e-9;
    twist_FET_tfall = 9e-9;

    twist_FET_Psw = 1/2*VHigh*ILow*twist_freq_switching*(twist_FET_trise + twist_FET_tfall);
end

== matlab function MMC_phase_hackathon_consensus_PWM_JABBAR_20260927/ /Subsystem/Subsystem/Hardware M5/Power losses branch 2/Branch DT loss ==
  data: twist_FET_Pdt output; ILow input
function twist_FET_Pdt = powerLossesDeadTime(ILow)
    %Twist gate power losses
    twist_freq_switching = 200e3;
    twist_FET_Vf = 1.2;
    twist_FET_tDr = 10e-9;
    twist_FET_tDf = 0;

    twist_FET_Pdt = twist_FET_Vf*ILow*(twist_FET_tDr+twist_FET_tDf)*twist_freq_switching;
end

== matlab function MMC_phase_hackathon_consensus_PWM_JABBAR_20260927/ /Subsystem/Subsystem/Hardware M5/Power losses branch 2/Branch cond loss ==
  data: twist_FET_Pcond output; VHigh input; VLow input; ILow input
function twist_FET_Pcond = powerLossesCond(VHigh, VLow, ILow)
    %Twist conduction power losses
    twist_FET_Ron = 0.025;

    twist_FET_PcondH = pow2(ILow)*twist_FET_Ron*(VLow/VHigh);
    twist_FET_PcondL = pow2(ILow)*twist_FET_Ron*(1 - VLow/VHigh);

    twist_FET_Pcond = twist_FET_PcondH + twist_FET_PcondL;
end

== matlab function MMC_phase_hackathon_consensus_PWM_JABBAR_20260927/ /Subsystem/Subsystem/Hardware M5/Power losses branch 2/Branch gate loss ==
  data: twist_FET_Pg output
function twist_FET_Pg = powerLossesGate()
    %Twist gate power losses
    twist_freq_switching = 200e3;
    twist_FET_QgH = 31e-9;
    twist_FET_QgL = 31e-9;
    twist_FET_Vgs = 11;

    twist_FET_Pg = (twist_FET_QgH + twist_FET_QgL)*twist_FET_Vgs*twist_freq_switching;
end

== matlab function MMC_phase_hackathon_consensus_PWM_JABBAR_20260927/ /Subsystem/Subsystem/Hardware M5/Power losses branch 2/Branch switching loss ==
  data: VHigh input; twist_FET_Psw output; ILow input
function twist_FET_Psw = powerLossesSwitch(VHigh, ILow)
    %Twist switch power losses
    twist_freq_switching = 200e3;
    twist_FET_trise = 17e-9;
    twist_FET_tfall = 9e-9;

    twist_FET_Psw = 1/2*VHigh*ILow*twist_freq_switching*(twist_FET_trise + twist_FET_tfall);
end

== matlab function MMC_phase_hackathon_consensus_PWM_JABBAR_20260927/ /Sinus Modulation + Sorting Algorithm/Subsystem1/Subsystem1/MATLAB Function1 ==
  data: Vc_arm input; i input; Vc_prev output; Vc_next output
function [Vc_prev, Vc_next] = get_neighbors(Vc_arm, i)
%#codegen
% Returns the capacitor voltages of the previous and next (circular) neighbors.
% Hardcoded strictly for N = 5 sub-modules per arm.

N = 5; 

% MATHEMATICAL CIRCULAR INDEXING FOR N = 5:
% If i=1 -> idx_prev = 5, idx_next = 2
% If i=5 -> idx_prev = 4, idx_next = 1

idx_prev = mod(i - 2, N) + 1;
idx_next = mod(i, N) + 1;

Vc_prev = Vc_arm(idx_prev);
Vc_next = Vc_arm(idx_next);

end

== matlab function MMC_phase_hackathon_consensus_PWM_JABBAR_20260927/ /Sinus Modulation + Sorting Algorithm/Subsystem1/Subsystem1/MATLAB Function3 ==
  data: sm_id input; m_arm input; gate_signal output; i_arm input; Vc_arm input; Vc_prev input; Vc_next input; N input
function gate_signal = hb_sm_local_ctrl_neighbor(sm_id, m_arm, i_arm, Vc_arm, Vc_prev, Vc_next, N)
%#codegen
% =========================================================
% LOCAL CONSENSUS BALANCING (v9) - matched to existing PSC-PWM hardware
%
% Implements the user's hb_sm_local_ctrl_consensus algorithm:
%   - Consensus balancing with neighbour-only Vref (distributed)
%   - Voltage deadband suppresses correction near steady state
%   - tanh(i_arm/Iscale) smooth sign avoids zero-current discontinuity
%
% Output is m_i as a continuous duty in [0, 1]. The downstream PWM
% Generator block carries the phase-shifted carrier (Phase = sps.Pc,
% configured per-SM in the parameter file) and produces the actual
% gate signal -- so we get phase-shifted PWM switching at the arm
% level without needing to generate a carrier in software.
%
% Inputs N and Vc_arm beyond v_current are unused but kept in the
% signature so the parent subsystem wiring is unchanged.
% =========================================================

% --- 1. PARAMETERS (verbatim from user spec) ---
k_v      = double(0.2);    % Balancing gain (1/V)
deadband = double(0.1);    % Voltage-error deadband (V)
Iscale   = double(1.0);    % Current scaling for tanh smoothing (A)

% --- 2. CONSENSUS BALANCING WITH LOCAL NEIGHBOUR REFERENCE ---
Vc_i = double(Vc_arm(sm_id));

% err: deviation of this SM from its immediate neighbours.
%   err > 0  -> this SM is BELOW neighbour average -> needs more charge
%   err < 0  -> this SM is ABOVE neighbour average -> needs less charge
err = double(0.5 * (Vc_prev + Vc_next)) - Vc_i;

% Deadband: ignore micro-imbalance near steady state.
if abs(err) < deadband
    err = 0.0;
end

% dir: smooth current-direction signal via tanh.
% Avoids the discontinuity of sign() near zero current crossings.
dir = tanh(double(i_arm) / Iscale);

% dm: balancing correction on the modulation index
dm = k_v * err * dir;

% m_i: per-SM corrected modulation index, clamped to [0, 1]
m_i = min(max(double(m_arm) + dm, 0.0), 1.0);

% --- 3. OUTPUT: duty cycle for the downstream phase-shifted PWM block ---
gate_signal = double(m_i);

end

== matlab function MMC_phase_hackathon_consensus_PWM_JABBAR_20260927/ /Subsystem/Subsystem1/Hardware M1/Feeder block/MATLAB Function ==
  data: i_feeder input; vC input; isfeederdisabled input; active_1 input; y output; Q_VCC output
function [y,Q_VCC]  = feeder_characteristics(i_feeder,vC,isfeederdisabled,active_1)

if(isfeederdisabled == 1)
    if(vC>=9.7)
        y = 11.2e-3;
        Q_VCC = 0;
    elseif(vC>=8.9 && vC < 9.7)
        if(active_1 == true)
            y = 11.2e-3;
            Q_VCC = 0;
        else
            y = 0;
            Q_VCC = 1;
        end
    else
        y = 0;
        Q_VCC = 1;
    end
else
    if(vC>=9.7)
        y = i_feeder;
        Q_VCC = 0;
    elseif(vC>=8.9 && vC < 9.7)
        if(active_1 == true)
            y = i_feeder;
            Q_VCC = 0;
        else
            y = 0;
            Q_VCC = 1;
        end
    else
        y = 0;
        Q_VCC = 1;
    end
end

== matlab function MMC_phase_hackathon_consensus_PWM_JABBAR_20260927/ /Subsystem/Subsystem1/Hardware M1/Power losses branch 1/Branch DT loss ==
  data: twist_FET_Pdt output; ILow input
function twist_FET_Pdt = powerLossesDeadTime(ILow)
    %Twist gate power losses
    twist_freq_switching = 200e3;
    twist_FET_Vf = 1.2;
    twist_FET_tDr = 10e-9;
    twist_FET_tDf = 0;

    twist_FET_Pdt = twist_FET_Vf*ILow*(twist_FET_tDr+twist_FET_tDf)*twist_freq_switching;
end

== matlab function MMC_phase_hackathon_consensus_PWM_JABBAR_20260927/ /Subsystem/Subsystem1/Hardware M1/Power losses branch 1/Branch cond loss ==
  data: twist_FET_Pcond output; VHigh input; VLow input; ILow input
function twist_FET_Pcond = powerLossesCond(VHigh, VLow, ILow)
    %Twist conduction power losses
    twist_FET_Ron = 0.025;

    twist_FET_PcondH = pow2(ILow)*twist_FET_Ron*(VLow/VHigh);
    twist_FET_PcondL = pow2(ILow)*twist_FET_Ron*(1 - VLow/VHigh);

    twist_FET_Pcond = twist_FET_PcondH + twist_FET_PcondL;
end

== matlab function MMC_phase_hackathon_consensus_PWM_JABBAR_20260927/ /Subsystem/Subsystem1/Hardware M1/Power losses branch 1/Branch gate loss ==
  data: twist_FET_Pg output
function twist_FET_Pg = powerLossesGate()
    %Twist gate power losses
    twist_freq_switching = 200e3;
    twist_FET_QgH = 31e-9;
    twist_FET_QgL = 31e-9;
    twist_FET_Vgs = 11;

    twist_FET_Pg = (twist_FET_QgH + twist_FET_QgL)*twist_FET_Vgs*twist_freq_switching;
end

== matlab function MMC_phase_hackathon_consensus_PWM_JABBAR_20260927/ /Subsystem/Subsystem1/Hardware M1/Power losses branch 1/Branch switching loss ==
  data: VHigh input; twist_FET_Psw output; ILow input
function twist_FET_Psw = powerLossesSwitch(VHigh, ILow)
    %Twist switch power losses
    twist_freq_switching = 200e3;
    twist_FET_trise = 17e-9;
    twist_FET_tfall = 9e-9;

    twist_FET_Psw = 1/2*VHigh*ILow*twist_freq_switching*(twist_FET_trise + twist_FET_tfall);
end

== matlab function MMC_phase_hackathon_consensus_PWM_JABBAR_20260927/ /Subsystem/Subsystem/Hardware M2/Power losses branch 1/Branch DT loss ==
  data: twist_FET_Pdt output; ILow input
function twist_FET_Pdt = powerLossesDeadTime(ILow)
    %Twist gate power losses
    twist_freq_switching = 200e3;
    twist_FET_Vf = 1.2;
    twist_FET_tDr = 10e-9;
    twist_FET_tDf = 0;

    twist_FET_Pdt = twist_FET_Vf*ILow*(twist_FET_tDr+twist_FET_tDf)*twist_freq_switching;
end

== matlab function MMC_phase_hackathon_consensus_PWM_JABBAR_20260927/ /Subsystem/Subsystem1/Hardware M1/Power losses branch 2/Branch DT loss ==
  data: twist_FET_Pdt output; ILow input
function twist_FET_Pdt = powerLossesDeadTime(ILow)
    %Twist gate power losses
    twist_freq_switching = 200e3;
    twist_FET_Vf = 1.2;
    twist_FET_tDr = 10e-9;
    twist_FET_tDf = 0;

    twist_FET_Pdt = twist_FET_Vf*ILow*(twist_FET_tDr+twist_FET_tDf)*twist_freq_switching;
end

== matlab function MMC_phase_hackathon_consensus_PWM_JABBAR_20260927/ /Subsystem/Subsystem1/Hardware M1/Power losses branch 2/Branch cond loss ==
  data: twist_FET_Pcond output; VHigh input; VLow input; ILow input
function twist_FET_Pcond = powerLossesCond(VHigh, VLow, ILow)
    %Twist conduction power losses
    twist_FET_Ron = 0.025;

    twist_FET_PcondH = pow2(ILow)*twist_FET_Ron*(VLow/VHigh);
    twist_FET_PcondL = pow2(ILow)*twist_FET_Ron*(1 - VLow/VHigh);

    twist_FET_Pcond = twist_FET_PcondH + twist_FET_PcondL;
end

== matlab function MMC_phase_hackathon_consensus_PWM_JABBAR_20260927/ /Subsystem/Subsystem1/Hardware M1/Power losses branch 2/Branch gate loss ==
  data: twist_FET_Pg output
function twist_FET_Pg = powerLossesGate()
    %Twist gate power losses
    twist_freq_switching = 200e3;
    twist_FET_QgH = 31e-9;
    twist_FET_QgL = 31e-9;
    twist_FET_Vgs = 11;

    twist_FET_Pg = (twist_FET_QgH + twist_FET_QgL)*twist_FET_Vgs*twist_freq_switching;
end
